simulink library "AFCToolbox2023a"  (R2023a)
settings: Solver=VariableStepAuto  StartTime=0.0  StopTime=10.0  RelTol=1e-3
undefined symbols (not defined in the file or in its folder): AFC5Toolbox_SimuMoudle, AFCToolbox, ax, ay, az, btnSample, C_d, C_dm, C_m, C_t, Control, d, declination_table, dp0, dp1, dp2, dp3, dt, euler_0, g0, I_xyz, inclination_table, J_m, lmd_high, lmd_low, lp_acc_knoise, lp_acc_max, lp_acc_min, lp_acc_seed, lp_GPS_BL_max, lp_GPS_BL_min, lp_GPS_H_max, lp_GPS_H_min, lp_GPS_knoise, lp_GPS_seed, lp_GPS_vel_max, lp_GPS_vel_min, lp_gyro_knoise, lp_gyro_max, lp_gyro_min, lp_gyro_seed, lp_hf_vwind, lp_hs_vwind_interp, lp_kaerorho, lp_kaeroT, lp_kIxyz, lp_kmass, lp_momentx_A0, lp_momentx_Af, lp_momentx_ts, lp_momenty_A0, lp_momenty_Af, lp_momenty_ts, lp_momentz_A0, lp_momentz_Af, lp_momentz_ts, lp_vf_vwind, lp_vs_vwind_interp, lp_vwind_thetax, lp_vwind_thetaz ... (+54)
libraries: $bdroot x104, simulink x75, etargetslib x32, sharedtransform x13, simulink_extras x12, dspstat3 x11, aerolibconvert2 x9, aerolibtransform2 x3, aerolibutil x2, matrix_library x1
(part 1 of 10)
settings Model: Creator=Brolian  LastModifiedBy=zqhkd
settings SolverCC: AlgebraicLoopSolver=TrustRegion
settings DataIOCC: ReturnWorkspaceOutputs=off
settings DebuggingCC: UnconnectedInputMsg=warning  UnconnectedOutputMsg=warning  UnconnectedLineMsg=warning  ArithmeticOperatorsInVariantConditions=warning
settings ModelReferenceCC: EnableRefExpFcnMdlSchedulingChecks=on
settings SFSimCC: SimUseLocalCustomCode=off  CustomCodeUndefinedFunction=UseInterfaceOnly
settings RTWCC: RTWUseLocalCustomCode=off
settings CodeAppCC: StateflowObjectComments=on
settings ConfigComp: CovBoundaryAbsTol=1.0e-5

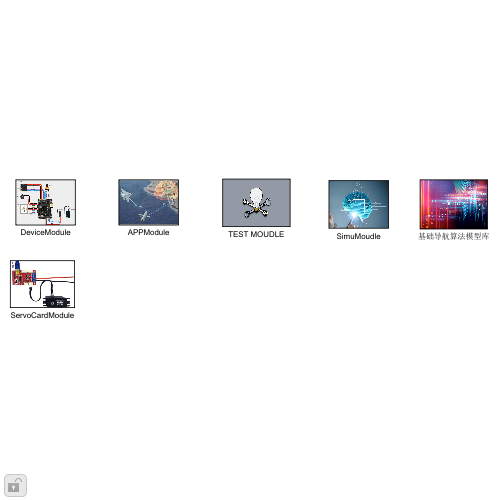
[thumbnail: Simulink's stored preview of the top-level diagram]
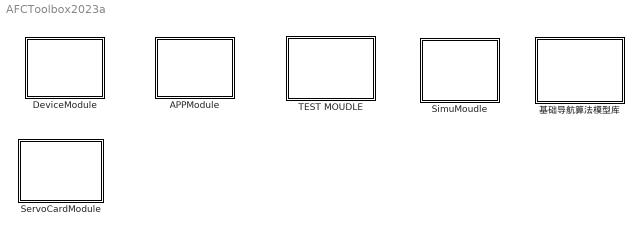
== system AFCToolbox2023a ==
  APPModule : Subsystem
      mask Display: image('AFCApp.png'); % 使用工具条上的 "编辑图像" 进行更改。
  DeviceModule : Subsystem
      mask Display: image('AFCDevice.png'); % 使用工具条上的 "编辑图像" 进行更改。
  ServoCardModule : Subsystem
      mask Display: image('ACEServoCard.png');
  SimuMoudle : Subsystem
      mask Display: image('SimuModule.png'); % 使用工具条上的 "编辑图像" 进行更改。
  TEST MOUDLE : Subsystem
      mask Display: image('TestModule.png'); % 使用工具条上的 "编辑图像" 进行更改。
  基础导航算法模型库 : Subsystem
      mask Display: image('AlgModule.png'); % 使用工具条上的 "编辑图像" 进行更改。

== system AFCToolbox2023a/APPModule ==
  note: ahrs和takeOffLand为V5.03以前
      | 版本库模块，由于Wxyz、Axyz
      | 采用地址传递方式，进行安装正
      | 负号反向处理时已被RTW优化掉
  AFC5StsBit : Subsystem
  RCLimit : S-Function  Priority=4  FunctionName=rcLimitAPI  Parameters=0  SFunctionDeploymentMode=off  EnableBusSupport=off  mask{g_pv=0}
      mask DialogControl Container1 Prompt: AFC-5无人机限幅模块
      mask Display:
      | color('gray');port_label('input',1,'bRCRollLT1000');
      | color('gray');port_label('input',2,'bRCPitchLT1000');
      | color('gray');port_label('input',3,'bRCThrottleEQ0');
      | color('gray');port_label('input',4,'bRCCh3CmdLT1400');
      | color('gray');port_label('input',5,'bRCCh2CmdLT1400');
      | color('gray');port_label('input',6,'bRCCh1CmdLT1600');
      | color('gray');port_label('input',7,'bRCCh0CmdLT1600');
  ahrs : S-Function  Priority=3  Commented=on  FunctionName=ahrsAPI  Parameters=0  SFunctionDeploymentMode=off  EnableBusSupport=off  mask{kp=0.14, ki=0.0087, kp_yaw=0.16, ki_yaw=0.001, dt=0.002, g=9.80665}
      mask prompts: kp "比例控制参数"; ki "积分控制参数"; kp_yaw "比例控制参数"; ki_yaw "积分控制参数"; dt "时间参数"; g "重力加速度"
      mask DialogControl DescGroupVar Prompt: 角速率PI控制参数输入窗口
      mask DialogControl Container2 Prompt: 偏航角速率PI控制参数输入窗口
      mask DialogControl Container3 Prompt: 参数设置窗口
      mask Display:
      | color('gray');port_label('input',1,'Wxyz');
      | color('gray');port_label('input',2,'Axyz');
      | color('gray');port_label('input',3,'HeadAng');
      | color('gray');port_label('input',4,'FastSts');
      | color('gray');port_label('output',1,'dcmAng');
      | color('gray');port_label('output',2,'dcmWxyz');
  ahrsN : S-Function  Priority=3  FunctionName=ahrsNAPI  Parameters=0  SFunctionDeploymentMode=off  EnableBusSupport=off  mask{kp=0.14, ki=0.0087, kp_yaw=0.16, ki_yaw=0.001, dt=0.002, g=9.80665}
      mask prompts: kp "比例控制参数"; ki "积分控制参数"; kp_yaw "比例控制参数"; ki_yaw "积分控制参数"; dt "时间参数"; g "重力加速度"
      mask DialogControl DescGroupVar Prompt: 角速率PI控制参数输入窗口
      mask DialogControl Container2 Prompt: 偏航角速率PI控制参数输入窗口
      mask DialogControl Container3 Prompt: 参数设置窗口
      mask Display:
      | color('gray');port_label('input',1,'Wx /rad/s');
      | color('gray');port_label('input',2,'Wy /rad/s');
      | color('gray');port_label('input',3,'Wz /rad/s');
      | color('gray');port_label('input',4,'Ax /m/s^2');
      | color('gray');port_label('input',5,'Ay /m/s^2');
      | color('gray');port_label('input',6,'Az /m/s^2');
      | color('gray');port_label('input',7,'HeadAng /°');
      | color('gray');port_label('input',8,'FastSts');
      | color('gray');port_label('output',1,'dcmAng /rad');
      | color('gray');port_label('output',2,'dcmWxyz /rad/s');
  altThrottle : S-Function  Priority=4  FunctionName=altThrottleAPI  Parameters=0  SFunctionDeploymentMode=off  EnableBusSupport=off
      mask DialogControl g_pv Prompt: 根据高度通道参数计算油门大小
      mask Display:
      | color('gray');port_label('input',1,'AFC5Sts');
      | color('gray');port_label('input',2,'PosZ');
      | color('gray');port_label('input',3,'VelZ');
      | color('gray');port_label('input',4,'ClimbRate');
      | color('gray');port_label('input',5,'dcmRoll');
      | color('gray');port_label('input',6,'dcmPitch');
      | color('gray');port_label('input',7,'altAccInt');
      | color('gray');port_label('input',8,'posTarZ');
      | color('gray');port_label('input',9,'ThrotHover');
      | color('gray');port_label('output',1,'Throttle');
  altitude : S-Function  Priority=3  FunctionName=altitudeAPI  Parameters=0  SFunctionDeploymentMode=off  EnableBusSupport=off  mask{alt_pos_kp=1.8, pid_alt_rate_kp=8.0, pid_alt_rate_ki=0.1, pid_alt_rate_kd=1.0, pid_alt_rate_imax=800.0, pid_alt_accel_kp=1.36, pid_alt_accel_ki=0.1, pid_alt_accel_kd=0.08, pid_alt_accel_imax=800.0, k1=0.6, k2=0.12, k3=0.008, control_dt=0.002, g=9.80665}
      mask prompts: alt_pos_kp "比例系数"; pid_alt_rate_kp "比例系数"; pid_alt_rate_ki "积分系数"; pid_alt_rate_kd "微分系数"; pid_alt_rate_imax "积分系数最大值"; pid_alt_accel_kp "比例系数"; pid_alt_accel_ki "积分系数"; pid_alt_accel_kd "微分系数"; pid_alt_accel_imax "积分系数最大值"; k1 "位置更新系数"; k2 "速度更新系数"; k3 "加速度更新系数"; control_dt "姿态控制周期"; g "重力加速度"
      mask DialogControl DescGroupVar Prompt: 高度控制参数输入窗口
      mask DialogControl Container2 Prompt: 高度控制回路的位置系数
      mask DialogControl Container3 Prompt: 高度控制回路的速率系数
      mask DialogControl Container4 Prompt: 高度控制回路的加速度系数
      mask DialogControl Container5 Prompt: 高度更新系数输入窗口
      mask DialogControl Container6 Prompt: 参数设置输入窗口
      mask Display:
      | color('gray');port_label('input',1,'AFC5Sts');
      | color('gray');port_label('input',2,'Height /cm');
      | color('gray');port_label('input',3,'dcmRoll /rad');
      | color('gray');port_label('input',4,'dcmPitch /rad');
      | color('gray');port_label('input',5,'Throttle');
      | color('gray');port_label('output',1,'PosZ /cm');
      | color('gray');port_label('output',2,'VelZ /cm/s');
      | color('gray');port_label('output',3,'ThroHover');
  altitudeThrottle : S-Function  Priority=4  FunctionName=altitudeThrottleAPI  Parameters=0  SFunctionDeploymentMode=off  EnableBusSupport=off
      mask DialogControl g_pv Prompt: 根据高度通道参数计算油门大小
      mask Display:
      | color('gray');port_label('input',1,'AFC5Sts');
      | color('gray');port_label('input',2,'PosZ');
      | color('gray');port_label('input',3,'VelZ');
      | color('gray');port_label('input',4,'ClimbRate');
      | color('gray');port_label('input',5,'dcmRoll');
      | color('gray');port_label('input',6,'dcmPitch');
      | color('gray');port_label('input',7,'ThrotHover');
      | color('gray');port_label('output',1,'Throttle');
  attitudePos : S-Function  Priority=3  FunctionName=attitudePosAPI  Parameters=0  SFunctionDeploymentMode=off  EnableBusSupport=off
      mask DialogControl ParameterGroupVar Prompt: 参数
      mask Display:
      | color('gray');port_label('input',1,'rollCmd');
      | color('gray');port_label('input',2,'pitchCmd');
      | color('gray');port_label('input',3,'yawCmd');
      | color('gray');port_label('input',4,'dcmAng');
      | color('gray');port_label('input',5,'Wz');
      | color('gray');port_label('input',6,'AngEfTarZ');
      | color('gray');port_label('output',1,'RateBfTar');
      | color('gray');port_label('output',2,'AngEfTarZ');
  attitudeRate : S-Function  Priority=4  FunctionName=attitudeRateAPI  Parameters=0  SFunctionDeploymentMode=off  EnableBusSupport=off  mask{angle_kp0=8.0, angle_kp1=6.6, angle_kp2=8.0, pid_rate0_kp=0.32, pid_rate0_ki=0.1, pid_rate0_kd=3.5, pid_rate1_kp=0.32, pid_rate1_ki=0.1, pid_rate1_kd=3.5, pid_rate2_kp=0.6, pid_rate2_ki=0.03, pid_rate2_kd=1.5, pid_rate0_imax=500.0, pid_rate1_imax=500.0, pid_rate2_imax=500.0, max0=5000.0, min0=-5000.0, max1=5000.0, min1=-5000.0, max2=4000.0, min2=-4000.0, control_dt=0.002}
      mask prompts: angle_kp0 "横滚角比例系数"; angle_kp1 "俯仰角比例系数"; angle_kp2 "航向角比例系数"; pid_rate0_kp "比例系数"; pid_rate0_ki "积分系数"; pid_rate0_kd "微分系数"; pid_rate1_kp "比例系数"; pid_rate1_ki "积分系数"; pid_rate1_kd "微分系数"; pid_rate2_kp "比例系数"; pid_rate2_ki "积分系数"; pid_rate2_kd "微分系数"; pid_rate0_imax "横滚角速率积分系数最大值"; pid_rate1_imax "俯仰角速率积分系数最大值"; pid_rate2_imax "航向角速率积分系数最大值"; max0 "最大值"; min0 "最小值"; max1 "最大值"; min1 "最小值"; max2 "最大值"; min2 "最小值"; control_dt "姿态控制周期"
      mask DialogControl DescGroupVar Prompt: 姿态角初始化比例系数输入窗口
      mask DialogControl Container2 Prompt: 姿态角速率初始化PI参数输入窗口
      mask DialogControl Container3 Prompt: 横滚角PI参数
      mask DialogControl Container4 Prompt: 俯仰角PI参数
      mask DialogControl Container5 Prompt: 航向角PI参数
      mask DialogControl Container6 Prompt: 姿态角速率积分系数的最大值
      mask DialogControl Container8 Prompt: 姿态角输出限幅设置窗口
      mask DialogControl Container9 Prompt: 横滚角输出限幅
      mask DialogControl Container10 Prompt: 俯仰角输出限幅
      mask DialogControl Container11 Prompt: 航向角输出限幅
      mask DialogControl Container7 Prompt: 参数设置输入窗口
      mask Display:
      | color('gray');port_label('input',1,'AFC5Sts');
      | color('gray');port_label('input',2,'rateBfTar');
      | color('gray');port_label('input',3,'dcmWxyz');
      | color('gray');port_label('output',1,'ServOut');
  ctrlChCmdAPI : S-Function  Priority=3  FunctionName=ctrlChCmdAPI  Parameters=0  SFunctionDeploymentMode=off  EnableBusSupport=off
      mask DialogControl g_pv Prompt: 遥控器SBus原始指令转换为通道指令
      mask Display:
      | color('gray');port_label('input',1,'RCRaw');
      | color('gray');port_label('output',1,'CHCmd');
  flyModeRun : S-Function  Priority=4  FunctionName=flyModeRunAPI  Parameters=0  SFunctionDeploymentMode=off  EnableBusSupport=off
      mask DialogControl g_pv Prompt: 飞行模式调度程序
      mask Display:
      | color('gray');port_label('input',1,'AFCSts');
      | color('gray');port_label('input',2,'PosZ /cm');
      | color('gray');port_label('input',3,'VelZ /cm/s');
      | color('gray');port_label('input',4,'dcmAng /rad');
      | color('gray');port_label('input',5,'dcmWxyz /rad/s');
      | color('gray');port_label('input',6,'ThroHover');
      | color('gray');port_label('input',7,'CHCtrlCmd');
      | color('gray');port_label('output',1,'Throttle');
      | color('gray');port_label('output',2,'RateBfTar');
  getAFCSts : S-Function  Priority=0  FunctionName=getAFCStsAPI  Parameters=g_sampleTime  SFunctionDeploymentMode=off  EnableBusSupport=off  mask{g_sampleTime=0.002}
      mask prompts: g_sampleTime "请输入采样时间："
      mask DialogControl DescGroupVar Prompt: AFC5系统状态
      mask DialogControl g_pv Prompt: 获取AFC5飞控状态，包括:
      mask DialogControl Control2 Prompt: D0：bSystemInitSts,D1：bLandComplete
      mask DialogControl Control3 Prompt: D2：bArmedEnable,D3：bDcmFast
      mask DialogControl Control4 Prompt: D4：bSdCardWriteErr
      mask DialogControl Control5 Prompt: D8--D15：iTaskOverTimeNo
      mask Display: color('gray');port_label('output',1,'AFCSts');
  getRCCmd : S-Function  Commented=on  FunctionName=getRCCmdAPI  Parameters=0  SFunctionDeploymentMode=off  EnableBusSupport=off
      mask DialogControl g_pv Prompt: 通道指令输入模块
      mask Display:
      | color('gray');port_label('output',1,'RollSrvo');
      | color('gray');port_label('output',2,'PitchSrvo');
      | color('gray');port_label('output',3,'YawSrvo');
      | color('gray');port_label('output',4,'Throttle');
      | color('gray');port_label('output',5,'ClimbRate');
  groundProc : S-Function  Priority=4  FunctionName=groundProcAPI  Parameters=0  SFunctionDeploymentMode=off  EnableBusSupport=off
      mask DialogControl ParameterGroupVar Prompt: 参数
      mask Display:
      | color('gray');port_label('input',1,'PosZ');
      | color('gray');port_label('input',2,'dcmAng');
      | color('gray');port_label('input',3,'Wxyz');
      | color('gray');port_label('output',1,'angEfTarZ');
      | color('gray');port_label('output',2,'rateBfTar');
      | color('gray');port_label('output',3,'Throttle');
  initTakeOff : S-Function  Priority=5  FunctionName=initTakeOffAPI  Parameters=0  SFunctionDeploymentMode=off  EnableBusSupport=off
      mask DialogControl g_pv Prompt: 初始化起飞模块
      mask Display:
      | color('gray');port_label('input',1,'PosZ');
      | color('gray');port_label('input',2,'Throttle');
  motorsSlow : S-Function  Commented=on  FunctionName=motorsSlowAPI  Parameters=0  SFunctionDeploymentMode=off  EnableBusSupport=off
      mask DialogControl ParameterGroupVar Prompt: 参数
      mask Display:
      | color('gray');port_label('input',1,'AFC5Sts');
      | color('gray');port_label('input',2,'Throttle');
      | color('gray');port_label('input',3,'inMaxThrottle');
      | color('gray');port_label('output',1,'MaxThrottle');
  outMotorsVal : S-Function  Priority=5  FunctionName=outMotorsValAPI  Parameters=0  SFunctionDeploymentMode=off  EnableBusSupport=off
      mask DialogControl g_pv Prompt: 输出电机电调指令值模块
      mask Display:
      | color('gray');port_label('input',1,'AFC5Sts');
      | color('gray');port_label('input',2,'ServOut');
      | color('gray');port_label('input',3,'Throttle');
      | color('gray');port_label('output',1,'EscVal');
  takeOffLand : S-Function  Priority=5  Commented=on  FunctionName=takeOffLandAPI  Parameters=0  SFunctionDeploymentMode=off  EnableBusSupport=off  mask{RC_Climb_Rate=0}
      mask prompts: RC_Climb_Rate "攀爬速度阈值"
      mask DialogControl g_pv Prompt: 起飞着陆模块
      mask DialogControl Control1 Prompt: (在此添加文本)处理起飞前的IMU校准、遥控解锁，着陆标志判定，电机关机锁定等操作
      mask DialogControl Container2 Prompt: 起飞条件
      mask Display:
      | color('gray');port_label('input',1,'Wxyz');
      | color('gray');port_label('input',2,'Axyz');
      | color('gray');port_label('input',3,'dcmRoll');
      | color('gray');port_label('input',4,'dcmPitch');
      | color('gray');port_label('input',5,'Throttle');
  takeOffLandN : S-Function  Priority=5  FunctionName=takeOffLandNAPI  Parameters=0  SFunctionDeploymentMode=off  EnableBusSupport=off  mask{RC_Climb_Rate=0}
      mask prompts: RC_Climb_Rate "攀爬速度阈值"
      mask DialogControl g_pv Prompt: 起飞着陆模块
      mask DialogControl Control1 Prompt: (在此添加文本)处理起飞前的IMU校准、遥控解锁，着陆标志判定，电机关机锁定等操作
      mask DialogControl Container2 Prompt: 起飞条件
      mask Display:
      | color('gray');port_label('input',1,'Wx');
      | color('gray');port_label('input',2,'Wy');
      | color('gray');port_label('input',3,'Wz');
      | color('gray');port_label('input',4,'Ax');
      | color('gray');port_label('input',5,'Ay');
      | color('gray');port_label('input',6,'Az');
      | color('gray');port_label('input',7,'dcmRoll');
      | color('gray');port_label('input',8,'dcmPitch');
      | color('gray');port_label('input',9,'Throttle');
  u16Toi16 : S-Function  FunctionName=u16Toi16API  Parameters=0  SFunctionDeploymentMode=off  EnableBusSupport=off
      mask DialogControl ParameterGroupVar Prompt: 参数
      mask Display:
      | color('gray');port_label('input',1,'u16');
      | color('gray');port_label('output',1,'i16');
  u32Toi32 : S-Function  FunctionName=u32Toi32API  Parameters=0  SFunctionDeploymentMode=off  EnableBusSupport=off
      mask DialogControl ParameterGroupVar Prompt: 参数
      mask Display:
      | color('gray');port_label('input',1,'u32');
      | color('gray');port_label('output',1,'i32');
  u8Toi8 : S-Function  FunctionName=u8Toi8API  Parameters=0  SFunctionDeploymentMode=off  EnableBusSupport=off
      mask DialogControl ParameterGroupVar Prompt: 参数
      mask Display:
      | color('gray');port_label('input',1,'u8');
      | color('gray');port_label('output',1,'i8');
  updateCd : Subsystem  Commented=on  TreatAsAtomicUnit=on
      settings: MinAlgLoopOccurrences=on  RTWFileNameOpts=Use function name
      mask DialogControl DescGroupVar Prompt: update_cd_values
      mask DialogControl DescTextVar Prompt: 角度角速度单位从弧度转换为度*100

== system AFCToolbox2023a/DeviceModule ==
  AFCTimer : S-Function  Priority=0  FunctionName=sysTimerAPI  Parameters=g_sampleTime,g_comPort,g_instName,g_id  SFunctionDeploymentMode=off  EnableBusSupport=off  mask{g_sampleTime=0.002, g_comPort=6, g_instName=0, g_id=0}
      mask prompts: g_sampleTime "请输入采样时间："
      mask DialogControl DescGroupVar Prompt: AFC-5飞控快速原型时钟模块
      mask DialogControl Control2 Prompt: 本模块能够直接访问AFC-5飞控系统的运行时钟，单位为秒。
      mask Display: color('gray');port_label('output',1,'Tim');
  AdSample : S-Function  Priority=1  FunctionName=adSampleAPI  Parameters=g_sampleTime,g_comPort,g_instName,g_id  SFunctionDeploymentMode=off  EnableBusSupport=off  mask{g_sampleTime=0.01, g_comPort=0, g_instName=0, g_id=0}
      mask prompts: g_sampleTime "请输入采样时间(s)："; g_comPort "COMPORT"
      mask DialogControl DescGroupVar Prompt: 外部电压采集模块
      mask Display:
      | color('gray');port_label('output',1,'Tim /ms');
      | color('gray');port_label('output',2,'I  /A');
      | color('gray');port_label('output',3,'V  /V');
  ComXIn : S-Function  Priority=2  FunctionName=readXXXComAPI  Parameters=g_sampleTime,g_comPort,g_baudRate,g_dataSize,g_dataBits,g_parity,g_stopBits  SFunctionDeploymentMode=off  EnableBusSupport=off  mask{g_sampleTime=0.01, g_comPort=UART4(TTL), g_baudRate=115200, g_dataSize=1, g_dataBits=8, g_parity=0, g_stopBits=1}
      mask prompts: g_sampleTime "采样时间(s)："; g_comPort "请选择串口："; g_baudRate "波特率："; g_dataSize "帧字节数："; g_dataBits "数据位："; g_parity "校验位："; g_stopBits "停止位："
      mask TypeOptions g_comPort: UART4(TTL) | UART5(RS422) | UART6(TTL) | UART7(RS232) | UART8(RS232)
      mask DialogControl DescGroupVar Prompt: 数传串口输入模块
      mask DialogControl g_comPort Tooltip: 该帧类型码范围在80--90，且不同DtCom帧类型码不同
      mask Display:
      | comPort = get_param(gcb, 'g_comPort');
      | color('gray');port_label('output',1,comPort);
  ComXOut : S-Function  Priority=8  FunctionName=writeXXXComAPI  Parameters=g_comPort,g_baudRate,g_outFreq,g_dataBits,g_parity,g_stopBits  SFunctionDeploymentMode=off  EnableBusSupport=off  mask{g_comPort=UART4(TTL), g_baudRate=115200, g_outFreq=1, g_dataBits=8, g_parity=none, g_stopBits=1}
      mask prompts: g_comPort "请选择串口："; g_baudRate "波特率："; g_outFreq "该模块输出帧频次："; g_dataBits "数据位："; g_parity "校验位："; g_stopBits "停止位："
      mask TypeOptions g_comPort: UART4(TTL) | UART5(RS422) | UART6(TTL) | UART7(RS232) | UART8(RS232)
      mask DialogControl DescGroupVar Prompt: 数传串口输出模块
      mask DialogControl g_comPort Tooltip: 串口号
      mask DialogControl g_outFreq Tooltip: 仿真步长整数倍数，即多少个仿真步长输出一次帧数据
      mask Display:
      | comPort = get_param(gcb, 'g_comPort');
      | color('gray');port_label('input',1,comPort);
  DPS310 : S-Function  Priority=1  FunctionName=DPS310API  Parameters=g_sampleTime,g_comPort,g_instName,g_id  SFunctionDeploymentMode=off  EnableBusSupport=off  mask{g_sampleTime=0.01, g_comPort=6, g_instName=0, g_id=0}
      mask prompts: g_sampleTime "采样时间"
      mask DialogControl ParameterGroupVar Prompt: DPS310数字气压计模块
      mask DialogControl Control1 Prompt: 本模块能够读取数字气压计DPS310测得的压力、温度、气压高度
      mask Display:
      | color('gray');port_label('output',1,'Tim /ms');
      | color('gray');port_label('output',2,'Press /Pa');
      | color('gray');port_label('output',3,'Temp /°C');
      | color('gray');port_label('output',4,'BarHeight /m');
  DPS310Rst : Subsystem  Commented=on
  DTComIn : S-Function  Priority=2  FunctionName=readDtComAPI  Parameters=g_sampleTime,g_frameType,g_resFrameNum,g_comPort,g_instName,g_id  SFunctionDeploymentMode=off  EnableBusSupport=off  mask{g_sampleTime=0.01, g_frameType=20, g_resFrameNum=0, g_comPort=6, g_instName=0, g_id=0}
      mask prompts: g_sampleTime "采样时间(s)："; g_frameType "请输入帧类型码："; g_resFrameNum "请输入回令帧次数："
      mask DialogControl DescGroupVar Prompt: 数传串口输入模块
      mask DialogControl g_frameType Tooltip: 该帧类型码范围在80--90，且不同DtCom帧类型码不同
      mask DialogControl g_resFrameNum Tooltip: 当接收到本有效帧后，串口会中止当前发送，改为发送指定回令帧次数后恢复原发送操作，回令帧内容为串口输入时刻的时标和串口输入数据。
      mask DialogControl ChkDtComIn Prompt: 校验输入参数名称
      mask Display:
      | fno = get_param(gcb, 'g_frameType');
      | color('gray');port_label('output',1,'Tim');
      | color('gray');port_label('output',2,['readDT' newline '@' fno]);
  DTComOut : S-Function  Priority=8  FunctionName=writeDtComAPI  Parameters=g_frameType,g_outFreq,g_comPort,g_instName,g_id  SFunctionDeploymentMode=off  EnableBusSupport=off  mask{g_frameType=1, g_outFreq=1, g_comPort=0, g_instName=0, g_id=0}
      mask prompts: g_frameType "自定义帧类型码："; g_outFreq "该模块输出帧频次："
      mask DialogControl DescGroupVar Prompt: 数传串口输出模块
      mask DialogControl g_frameType Tooltip: 该帧类型码取值为1~20，且不同DtCom帧类型码不同
      mask DialogControl g_outFreq Tooltip: 仿真步长整数倍数，即多少个仿真步长输出一次帧数据
      mask DialogControl ChkSignalName Prompt: 校验信号名称
      mask Display:
      | fno = get_param(gcb, 'g_frameType');
      | color('gray');port_label('input',1,['writeDT@' fno]);
  DtOutDevParm : S-Function  FunctionName=DtOutDevParm  Parameters=g_bICM42688EO,g_bICM20602EO,g_bDPSISTEO,g_bGPSEO,g_bRemoterEO  SFunctionDeploymentMode=off  EnableBusSupport=off  mask{g_bICM42688EO=on, g_bICM20602EO=on, g_bDPSISTEO=on, g_bGPSEO=on, g_bRemoterEO=on}
      mask DialogControl ParameterGroupVar Prompt: 参数
  GPS : S-Function  Priority=1  FunctionName=readGpsAPI  Parameters=g_sampleTime,g_gpsDev,g_comPort,g_instName,g_id  SFunctionDeploymentMode=off  EnableBusSupport=off  mask{g_sampleTime=0.1, g_gpsDev=M10 GNSS, g_comPort=6, g_instName=0, g_id=0}
      mask prompts: g_sampleTime "请输入采样时间："; g_gpsDev "请选择GPS设备"
      mask TypeOptions g_gpsDev: M10 GNSS | NANO GNSS
      mask DialogControl DescGroupVar Prompt: GPS接收机信息获取模块
      mask DialogControl Control2 Prompt: 本模块能够直接读取如下GPS信息：Lat -- 纬度，北纬为正（单位：°）；Lon -- 经度，东经为正（单位：°），Alt -- 海拔高度（单位：m）Vx--M10表示正北速度、Nano-D表示ECCF坐标系下Vx（m/s），Vy--M10表示正东速度、Nano-D表示ECCF坐标系下Vy（m/s），Vz--M10表示向上速度、Nano-D表示ECCF坐标系下Vz（m/s），Vgnd -- 地速（单位：m/s），HeadAng -- 真北航向角（单位：°），STS -- GPS状态，stasN--卫星个数, hdop-- 水平精度因子
      mask DialogControl g_gpsDev Tooltip: 请通过下拉菜单选择指定GNSS设备
      mask Display:
      | color('gray');port_label('output',1,'GPSTim /s');
      | color('gray');port_label('output',2,'Lon /°');
      | color('gray');port_label('output',3,'Lat /°');
      | color('gray');port_label('output',4,'Alt /m');
      | color('gray');port_label('output',5,'Vx /m/s');
      | color('gray');port_label('output',6,'Vy /m/s');
      | color('gray');port_label('output',7,'Vz /m/s');
      | color('gray');port_label('output',8,'Vgnd /m/s');
      | color('gray');port_label('output',9,'Head /°');
      | color('gray');port_label('output',10,'Sts');
      | color('gray');port_label('output',11,'stasN');
      | color('gray');port_label('output',12,'hdop');
      | color('gray');port_label('output',13,'AFCTim /ms');
  GPUComIn : S-Function  Commented=on  FunctionName=readGpuComAPI  Parameters=g_frameType,g_sampleTime,g_comPort,g_instName,g_id  SFunctionDeploymentMode=off  EnableBusSupport=off  mask{g_frameType=162, g_sampleTime=0.01, g_comPort=0, g_instName=0, g_id=0}
      mask prompts: g_frameType "请输入帧类型码："; g_sampleTime "采样时间(s)："
      mask DialogControl DescGroupVar Prompt: 模型串口输入模块
      mask Display: color('gray');port_label('output',1,'readGPU');
  GPUComOut : S-Function  Commented=on  FunctionName=writeGpuComAPI  Parameters=g_frameType,g_comPort,g_instName,g_id  SFunctionDeploymentMode=off  EnableBusSupport=off  mask{g_frameType=2, g_comPort=0, g_instName=0, g_id=0}
      mask prompts: g_frameType "请输入帧类型码："
      mask DialogControl DescGroupVar Prompt: GPU串口输出模块
      mask Display: color('gray');port_label('input',1,'writeGPU');
  HiEscCmd : S-Function  Priority=6  FunctionName=hiEscCmdAPI  Parameters=g_chanelNo,g_minPW,g_maxPW,g_comPort,g_instName,g_id  SFunctionDeploymentMode=off  EnableBusSupport=off  mask{g_chanelNo=1, g_minPW=40, g_maxPW=80, g_comPort=6, g_instName=0, g_id=0}
      mask prompts: g_chanelNo "电调指令通道(1--12)："; g_minPW "电调指令最小值："; g_maxPW "电调指令最大值："; g_comPort "串行端口"; g_instName "实例名称"; g_id "ID号"
      mask DialogControl DescGroupVar Prompt: 进行高速电调控制指令参数配置
      mask DialogControl g_minPW Tooltip: 高速电调占空比最小值标称值为40%, 该值可根据实际情况做微小调整
      mask DialogControl g_maxPW Tooltip: 高速电调占空比最大值标称值为80%, 该值可根据实际情况做微小调整
      mask DialogControl Control1 Prompt: 高速电调频率为400Hz，电调指令输入值范围在0~100之间
      mask Display:
      | ch = get_param(gcb, 'g_chanelNo');
      | color('gray');port_label('input',1,['hiEsc#' ch]);
  ICM20602 : S-Function  Priority=0  FunctionName=ICM20602API  Parameters=g_sampleTime,g_GyroRangeSel,g_AcclRangeSel,g_smplrtDiv,g_comPort,g_instName,g_id  SFunctionDeploymentMode=off  EnableBusSupport=off  mask{g_sampleTime=0.002, g_GyroRangeSel=±2000 °/s, g_AcclRangeSel=±8g, g_smplrtDiv=0, g_comPort=6, g_instName=0, g_id=0}
      mask prompts: g_sampleTime "请输入采样时间："; g_GyroRangeSel "陀螺仪测量范围"; g_AcclRangeSel "加计测量范围"; g_smplrtDiv "采样速率分频："
      mask TypeOptions g_GyroRangeSel: ±250 °/s | ±500 °/s | ±1000 °/s | ±2000 °/s
      mask TypeOptions g_AcclRangeSel: ±2g | ±4g | ±8g | ±16g
      mask DialogControl DescGroupVar Prompt: ICM20602惯组接口模块
      mask DialogControl Control2 Prompt: 本模块能够读取ICM20602惯组模块的角速率（rad/s）、过载g（缺省为陀螺仪±250°/s, 加计±2g）
      mask Display:
      | color('gray');port_label('output',1,'Tim /ms');
      | color('gray');port_label('output',2,'Wx /°/s');
      | color('gray');port_label('output',3,'Wy /°/s');
      | color('gray');port_label('output',4,'Wz /°/s');
      | color('gray');port_label('output',5,'Ax / m/s^2');
      | color('gray');port_label('output',6,'Ay / m/s^2');
      | color('gray');port_label('output',7,'Az / m/s^2');
      | color('gray');port_label('output',8,'Temp /°');
  ICM42688 : S-Function  Priority=0  FunctionName=ICM42688API  Parameters=g_sampleTime,g_GyroRangeSel,g_AcclRangeSel,g_antiAliasFilter,g_notchFilter,g_comPort,g_instName,g_id  SFunctionDeploymentMode=off  EnableBusSupport=off  mask{g_sampleTime=0.002, g_GyroRangeSel=±2000 °/s, g_AcclRangeSel=±8g, g_antiAliasFilter=42, g_notchFilter=1449Hz, g_comPort=6, g_instName=0, g_id=0}
      mask prompts: g_sampleTime "请输入采样时间："; g_GyroRangeSel "陀螺仪测量范围"; g_AcclRangeSel "加计测量范围"; g_antiAliasFilter "抗混叠滤波器频率:"; g_notchFilter "限波器带宽:"; g_comPort "串口号"; g_instName "实例名"; g_id "ID号"
      mask TypeOptions g_GyroRangeSel: ±2000 °/s | ±1000°/s | ±500 °/s | ±250 °/s | ±125 °/s | ±62.5°/s | ±31.25°/s | ±15.625°/s
      mask TypeOptions g_AcclRangeSel: ±16g | ±8g | ±4g | ±2g
      mask TypeOptions g_antiAliasFilter: 禁止 | 42 Hz | 84 Hz | 126 Hz | 170 Hz | 213 Hz | 258 Hz | 303 Hz | 348 Hz | 394 Hz | 441 Hz | 488 Hz | 536 Hz | 585 Hz | 634 Hz | 684 Hz | 734 Hz | 785 Hz | 837 Hz | 890 Hz | 943 Hz | 997 Hz | 1051Hz | 1107Hz | 1163Hz | 1220Hz | 1277Hz | 1336Hz | 1395Hz | 1454Hz | 1515Hz | 1577Hz | 1639Hz | 1702Hz | 1766Hz | 1830Hz | 1896Hz | 1962Hz | 2029Hz | 2097Hz | 2166Hz | 2235Hz | 2306Hz | 2377Hz | 2449Hz | 2522Hz | 2596Hz | 2671Hz | 2746Hz | 2823Hz | 2900Hz | 2978Hz | 3057Hz | 3137Hz | 3217Hz | 3299Hz | 3381Hz | 3464Hz | 3548Hz | 3633Hz | 3718Hz | 3805Hz | 3892Hz | 3979Hz
      mask TypeOptions g_notchFilter: 禁止 | 1449Hz | 680  Hz | 329  Hz | 162  Hz | 80  Hz | 40  Hz | 20  Hz | 10  Hz
      mask DialogControl DescGroupVar Prompt: ICM42688惯组接口模块
      mask DialogControl Control2 Prompt: 本模块能够读取ICM42688惯组模块的角速率（rad/s）、过载g（缺省为陀螺仪±2000°/s, 加计±16g）
      mask DialogControl g_antiAliasFilter Tooltip: 可配置抗混叠滤波器频率为42~3979Hz
      mask DialogControl g_notchFilter Tooltip: 可配置限波器频率为10~1449Hz
      mask Display:
      | color('gray');port_label('output',1,'Tim /ms');
      | color('gray');port_label('output',2,'Wx /rad/s');
      | color('gray');port_label('output',3,'Wy /rad/s');
      | color('gray');port_label('output',4,'Wz /rad/s');
      | color('gray');port_label('output',5,'Ax /m/s^2');
      | color('gray');port_label('output',6,'Ay / m/s^2');
      | color('gray');port_label('output',7,'Az / m/s^2');
      | color('gray');port_label('output',8,'Temp /°');
  IST8310 : S-Function  Priority=1  FunctionName=IST8310API  Parameters=g_sampleTime,g_comPort,g_instName,g_id  SFunctionDeploymentMode=off  EnableBusSupport=off  mask{g_sampleTime=0.01, g_comPort=0, g_instName=0, g_id=0}
      mask prompts: g_sampleTime "请输入采样时间："
      mask DialogControl ParameterGroupVar Prompt: IST8310地磁传感器接口模块
      mask DialogControl Control1 Prompt: 本模块能够读取地磁传感器IST8310测得的三轴地磁强度（单位：uT）
      mask Display:
      | color('gray');port_label('output',1,'Tim /ms');
      | color('gray');port_label('output',2,'MagX /uT');
      | color('gray');port_label('output',3,'MagY /uT');
      | color('gray');port_label('output',4,'MagZ /uT');
      | color('gray');port_label('output',5,'HeadAng /°');
  LedBit : S-Function  Priority=6  FunctionName=ledBitAPI  Parameters=g_chanelNo,g_comPort,g_instName,g_id  SFunctionDeploymentMode=off  EnableBusSupport=off  mask{g_chanelNo=绿色指示灯, g_comPort=0, g_instName=0, g_id=0}
      mask prompts: g_chanelNo "指示灯："
      mask TypeOptions g_chanelNo: 黄色指示灯 | 绿色指示灯 | 蓝色指示灯 | 红色指示灯
      mask DialogControl DescGroupVar Prompt: 选择LED指示灯
      mask DialogControl g_chanelNo Tooltip: 请通过下拉菜单选择指定指示灯
      mask Display:
      | ch = get_param(gcb, 'g_chanelNo');
      | color('gray');port_label('input',1,ch);
      | %color('blue');
      | %disp(['MonitorIP' newline ch]);
      | %disp([newline newline ch]);
  LedGroup : S-Function  Priority=7  FunctionName=ledGroupAPI  Parameters=g_frameType,g_comPort,g_instName,g_id  SFunctionDeploymentMode=off  EnableBusSupport=off  mask{g_frameType=0, g_comPort=6, g_instName=0, g_id=0}
      mask prompts: g_frameType "请输入帧类型码："
      mask DialogControl DescGroupVar Prompt: LED颜色与系统状态指示模块
      mask Display:
      | color('gray');port_label('input',1,'Fly(Y)');
      | color('gray');port_label('input',2,'Test(G)');
      | color('gray');port_label('input',3,'DL(B)');
      | color('gray');port_label('input',4,'Err(R)');
  LowEscCmd : S-Function  Priority=6  FunctionName=lowEscCmdAPI  Parameters=g_chanelNo,g_minPW,g_maxPW,g_comPort,g_instName,g_id  SFunctionDeploymentMode=off  EnableBusSupport=off  mask{g_chanelNo=1, g_minPW=5.6, g_maxPW=11.45, g_comPort=6, g_instName=0, g_id=0}
      mask prompts: g_chanelNo "电调指令通道(1--12)："; g_minPW "电调指令最小值："; g_maxPW "电调指令最大值："; g_comPort "串行端口"; g_instName "实例名称"; g_id "ID号"
      mask DialogControl DescGroupVar Prompt: 进行低速电调控制指令参数配置
      mask DialogControl g_minPW Tooltip: 低速电调占空比最小值标称值为2.5%, 该值可根据实际情况做微小调整
      mask DialogControl g_maxPW Tooltip: 低速电调占空比最大值标称值为12.5%, 该值可根据实际情况做微小调整
      mask DialogControl Control1 Prompt: 低速电调频率为50Hz，电调指令输入值范围在0~100之间
      mask Display:
      | ch = get_param(gcb, 'g_chanelNo');
      | color('gray');port_label('input',1,['loEsc#' ch]);
  MS5525 : S-Function  Priority=1  FunctionName=MS5525API  Parameters=g_sampleTime,g_comPort,g_instName,g_id  SFunctionDeploymentMode=off  EnableBusSupport=off  mask{g_sampleTime=0.01, g_comPort=6, g_instName=0, g_id=0}
      mask prompts: g_sampleTime "采样时间"
      mask DialogControl ParameterGroupVar Prompt: MS5525空速计模块
      mask DialogControl Control1 Prompt: 本模块能够读取空速计MS5525测得的动压、温度和指示空速
      mask Display:
      | color('gray');port_label('output',1,'Tim /ms');
      | color('gray');port_label('output',2,'DifP /Pa');
      | color('gray');port_label('output',3,'Temp /°C');
      | color('gray');port_label('output',4,'IAS /m/s');
  MS5525Bias : S-Function  Priority=6  FunctionName=calMS5525BiasAPI  Parameters=g_sampleTime,g_comPort,g_instName,g_id  SFunctionDeploymentMode=off  EnableBusSupport=off  mask{g_sampleTime=2, g_comPort=0, g_instName=0, g_id=0}
      mask prompts: g_sampleTime "空速计校准采样时间（单位：秒）"
      mask DialogControl DescGroupVar Prompt: 空速计校准采样时间
      mask DialogControl g_sampleTime Tooltip: 请通过下拉菜单选择指定指示灯
      mask DialogControl Control1 Prompt: 【输入端口Calib接收到一个上升沿信号时执行校准操作】
      mask Display: color('gray');port_label('input',1,'Calib');
  PWMSample : S-Function  Priority=1  FunctionName=pwmSampleAPI  Parameters=g_sampleTime,g_comPort,g_instName,g_id  SFunctionDeploymentMode=off  EnableBusSupport=off  mask{g_sampleTime=0.01, g_comPort=6, g_instName=0, g_id=0}
      mask prompts: g_sampleTime "请输入采样时间(s)："
      mask DialogControl DescGroupVar Prompt: 舵系统角度采集模块
      mask DialogControl Control1 Prompt: 规定采样输出参数为-100~+100之间的值，其对应PWM 400Hz信号的高电平脉宽1ms~2ms, 占空比40%--80%
      mask Display:
      | color('gray');port_label('output',1,'Ch1');
      | color('gray');port_label('output',2,'Ch2');
  PressScanner : S-Function  Priority=1  FunctionName=pressScanAPI  Parameters=g_sampleTime,g_comPort,g_instName,g_id  SFunctionDeploymentMode=off  EnableBusSupport=off  mask{g_sampleTime=0.1, g_comPort=6, g_instName=0, g_id=0}
      mask prompts: g_sampleTime "请输入采样时间："
      mask DialogControl DescGroupVar Prompt: 压力扫描阀模块
      mask DialogControl Control2 Prompt: 本模块能够实时采集32通道压强信号。
      mask Display:
      | color('gray');port_label('output',1,'CH0 /kPa');
      | color('gray');port_label('output',2,'CH1 /kPa');
      | color('gray');port_label('output',3,'CH2 /kPa');
      | color('gray');port_label('output',4,'CH3 /kPa');
      | color('gray');port_label('output',5,'CH4 /kPa');
      | color('gray');port_label('output',6,'CH5 /kPa');
      | color('gray');port_label('output',7,'CH6 /kPa');
      | color('gray');port_label('output',8,'CH7 /kPa');
      | color('gray');port_label('output',9,'CH8 /kPa');
      | color('gray');port_label('output',10,'CH9 /kPa');
      | color('gray');port_label('output',11,'CH10 /kPa');
      | color('gray');port_label('output',12,'CH11 /kPa');
      | color('gray');port_label('output',13,'CH12 /kPa');
      | color('gray');port_label('output',14,'CH13 /kPa');
      | color('gray');port_label('output',15,'CH14 /kPa');
      | color('gray');port_label('output',16,'CH15 /kPa');
      | color('gray');port_label('output',17,'CH16 /kPa');
      | color('gray');port_label('output',18,'CH17 /kPa');
      | color('gray');port_label('output',19,'CH18 /kPa');
      | color('gray');port_label('output',20,'CH19 /kPa');
      | color('gray');port_label('output',21,'CH20 /kPa');
      | color('gray');port_label('output',22,'CH21 /kPa');
      | color('gray');port_label('output',23,'CH22 /kPa');
      | color('gray');port_label('output',24,'CH23 /kPa');
      | color('gray');port_label('output',25,'CH24 /kPa');
      | color('gray');port_label('output',26,'CH25 /kPa');
      | color('gray');port_label('output',27,'CH26 /kPa');
      | color('gray');port_label('output',28,'CH27 /kPa');
      | color('gray');port_label('output',29,'CH28 /kPa');
      | color('gray');port_label('output',30,'CH29 /kPa');
      | color('gray');port_label('output',31,'CH30 /kPa');
      | color('gray');port_label('output',32,'CH31 /kPa');
      | color('gray');port_label('output',33,'AFCTim /ms');
  SBusCmd : S-Function  Priority=0  FunctionName=readSBusCmdAPI  Parameters=g_sampleTime,g_chanelNo,g_comPort,g_instName,g_id  SFunctionDeploymentMode=off  EnableBusSupport=off  mask{g_sampleTime=0.002, g_chanelNo=1, g_comPort=6, g_instName=0, g_id=0}
      mask prompts: g_sampleTime "请输入采样时间(s)："; g_chanelNo "通道号："
      mask DialogControl DescGroupVar Prompt: 遥控指令采集模块
      mask DialogControl g_chanelNo Tooltip: 通道16为遥控指令刷新标志，其值为0表示未更新，1表示更新。
      mask DialogControl Control1 Prompt: 遥控器采集原始值，各通道原始值范围为352(0x160)--1695(0x69F)，中位1024(0x400)。
      mask Display: color('gray');port_label('output',1,'Cmd');
  SeqInst : S-Function  Priority=6  FunctionName=seqCtrlAPI  Parameters=g_chanelNo,g_comPort,g_instName,g_id  SFunctionDeploymentMode=off  EnableBusSupport=off  mask{g_chanelNo=时序指令1, g_comPort=0, g_instName=0, g_id=0}
      mask prompts: g_chanelNo "时序指令通道号："
      mask TypeOptions g_chanelNo: 时序指令1 | 时序指令2 | 时序指令3 | 时序指令4 | 时序指令5 | 时序指令6 | 时序指令7 | 时序指令8
      mask DialogControl DescGroupVar Prompt: 选择时序控制指令
      mask DialogControl g_chanelNo Tooltip: 请通过下拉菜单选择指定指示灯
      mask Display:
      | %color('gray');port_label('input',1,'S');
      | chNo = get_param(gcbh, 'g_chanelNo');
      | disp(chNo);
  SimuComIn : S-Function  Priority=2  FunctionName=readSimuComAPI  Parameters=g_sampleTime,g_frameType,g_resFrameNum,g_comPort,g_instName,g_id  SFunctionDeploymentMode=off  EnableBusSupport=off  mask{g_sampleTime=0.01, g_frameType=80, g_resFrameNum=0, g_comPort=6, g_instName=0, g_id=0}
      mask prompts: g_sampleTime "采样时间(s)："; g_frameType "请输入帧类型码："; g_resFrameNum "请输入回令帧帧数："
      mask DialogControl DescGroupVar Prompt: 仿真串口输入模块
      mask DialogControl g_frameType Tooltip: 自定义帧类型码范围在1--20，且不同SimuCom帧类型码不同
      mask DialogControl g_resFrameNum Tooltip: 当接收到本有效帧后，串口会中止当前发送，改为发送指定回令帧次数后恢复原发送操作，回令帧内容为串口输入时刻的时标和串口输入数据。
      mask Display:
      | color('gray');port_label('output',1,'Tim');
      | color('gray');port_label('output',2,'readSimu');
  SimuComOut : S-Function  Priority=8  FunctionName=writeSimuComAPI  Parameters=g_frameType,g_outFreq,g_comPort,g_instName,g_id  SFunctionDeploymentMode=off  EnableBusSupport=off  mask{g_frameType=1, g_outFreq=1, g_comPort=0, g_instName=0, g_id=0}
      mask prompts: g_frameType "请输入帧类型码："; g_outFreq "该模块输出帧频次："
      mask DialogControl DescGroupVar Prompt: 仿真串口输出模块
      mask DialogControl g_frameType Tooltip: 该帧类型码取值为1~20，且不同SimuCom帧类型码不同
      mask DialogControl g_outFreq Tooltip: 仿真步长整数倍数，即多少个仿真步长输出一次帧数据
      mask Display: color('gray');port_label('input',1,'writeSimu');
  SrvoCmd : S-Function  Commented=on  FunctionName=srvoCmdAPI  Parameters=g_chanelNo,g_minPW,g_maxPW,g_comPort,g_instName,g_id  SFunctionDeploymentMode=off  EnableBusSupport=off  mask{g_chanelNo=1, g_minPW=40, g_maxPW=76.72, g_comPort=0, g_instName=0, g_id=0}
      mask prompts: g_chanelNo "舵机指令通道(1--12)："; g_minPW "最小开度占空比%："; g_maxPW "最大开度占空比%："
      mask DialogControl DescGroupVar Prompt: 进行舵机控制指令参数配置
      mask DialogControl g_minPW Tooltip: 值在2--90之间，需要用示波器监测
      mask DialogControl g_maxPW Tooltip: 值在2--90之间，需要用示波器监测
      mask DialogControl Control1 Prompt: 舵机指令输入值范围为-90~+90
      mask Display: color('gray');port_label('input',1,'Inst');
  StartSts : S-Function  Priority=2  AncestorBlock=AFCToolbox/btnSample  FunctionName=startStsSampleAPI  Parameters=g_sampleTime,g_comPort,g_instName,g_id  SFunctionDeploymentMode=off  EnableBusSupport=off  mask{g_sampleTime=0.01, g_comPort=0, g_instName=0, g_id=0}
      mask prompts: g_sampleTime "请输入采样时间(s)："
      mask DialogControl DescGroupVar Prompt: 启动开关或同步开关状态采集模块
      mask Display: color('gray');port_label('output',1,'Start');
  TF03 : S-Function  Priority=1  FunctionName=TOF03API  Parameters=g_sampleTime,g_slideNum,g_comPort,g_instName,g_id  SFunctionDeploymentMode=off  EnableBusSupport=off  mask{g_sampleTime=0.01, g_slideNum=1, g_comPort=0, g_instName=0, g_id=0}
      mask prompts: g_sampleTime "请输入采样时间(s)："; g_slideNum "滑动滤波数据点数："; g_comPort "COMPORT"
      mask DialogControl DescGroupVar Prompt: 激光测距TF03模块
      mask DialogControl Control1 Prompt: 该模块输出激光测距值，最大测量范围0.1m--100m/180m, 测量精度10cm，和信号强度，正常测距的信号强度值范围为40--1200，低于40测距超量程
      mask Display:
      | color('gray');port_label('output',1,'Tim /ms');
      | color('gray');port_label('output',2,'Dist /m');
      | color('gray');port_label('output',3,'Strg');
  TaskScheduler : S-Function  Priority=2  FunctionName=taskSchedulerAPI  Parameters=task01Period,task02Period,task03Period  SFunctionDeploymentMode=off  EnableBusSupport=off  mask{task01Period=10, task02Period=0, task03Period=0}
      mask prompts: task01Period "Task01高优先级任务周期(ms)："; task02Period "Task02高优先级任务周期(ms)："; task03Period "Task03高优先级任务周期(ms)："
      mask DialogControl DescGroupVar Prompt: 任务调度模块
      mask DialogControl task01Period Tooltip: 设置为0时将关闭该任务线程
      mask DialogControl task02Period Tooltip: 设置为0时将关闭该任务线程
      mask DialogControl task03Period Tooltip: 设置为0时将关闭该任务线程
      mask Display: color('gray');port_label('output',1,'Task');
  TempratureScanner : S-Function  Priority=1  FunctionName=tempratureScanAPI  Parameters=g_sampleTime,g_comPort,g_instName,g_id  SFunctionDeploymentMode=off  EnableBusSupport=off  mask{g_sampleTime=0.1, g_comPort=6, g_instName=0, g_id=0}
      mask prompts: g_sampleTime "请输入采样时间："
      mask DialogControl DescGroupVar Prompt: 温度扫描阀模块
      mask DialogControl Control2 Prompt: 本模块能够实时采集12通道温度信号。
      mask Display:
      | color('gray');port_label('output',1,'CH0 /°C');
      | color('gray');port_label('output',2,'CH1 /°C');
      | color('gray');port_label('output',3,'CH2 /°C');
      | color('gray');port_label('output',4,'CH3 /°C');
      | color('gray');port_label('output',5,'CH4 /°C');
      | color('gray');port_label('output',6,'CH5 /°C');
      | color('gray');port_label('output',7,'CH6 /°C');
      | color('gray');port_label('output',8,'CH7 /°C');
      | color('gray');port_label('output',9,'CH8 /°C');
      | color('gray');port_label('output',10,'CH9 /°C');
      | color('gray');port_label('output',11,'CH10 /°C');
      | color('gray');port_label('output',12,'CH11 /°C');
      | color('gray');port_label('output',13,'AFCTim /ms');
  USBDisk : S-Function  Priority=8  FunctionName=writeUSBDiskAPI  Parameters=g_taskName,g_varName,g_outFreq,g_comPort,g_instName,g_id  SFunctionDeploymentMode=off  EnableBusSupport=off  mask{g_taskName=F, g_varName=x1,x2,x3,x4, g_outFreq=1, g_comPort=0, g_instName=0, g_id=0}
      mask prompts: g_taskName "请输入任务名称："; g_varName "请输入用逗号分开的所有变量名称："; g_outFreq "请输入写入频次："
      mask DialogControl DescGroupVar Prompt: USB DISK存盘模块
      mask DialogControl g_taskName Tooltip: 任务名长度不超过8个字符
      mask DialogControl g_varName Tooltip: 该名称为数据首行的抬头
      mask DialogControl g_outFreq Tooltip: 写入频次应该为仿真步长整数倍，如果为0表示不写入
      mask Display: color('gray');port_label('input',1,'writeDisk');
  UavId : S-Function  Priority=0  FunctionName=uavIdAPI  Parameters=g_sampleTime,g_comPort,g_instName,g_id  SFunctionDeploymentMode=off  EnableBusSupport=off  mask{g_sampleTime=0.002, g_comPort=6, g_instName=0, g_id=0}
      mask prompts: g_sampleTime "请输入采样时间："
      mask DialogControl DescGroupVar Prompt: AFC-5飞控组件ID获取模块
      mask DialogControl Control2 Prompt: 本模块能够直接读取AFC-5飞控组件ID号
      mask Display: color('gray');port_label('output',1,'uavID');
  UserEscCmd : S-Function  Priority=6  FunctionName=userEscCmdAPI  Parameters=g_chanelNo,g_minPW,g_maxPW,g_userFreq,g_comPort,g_instName,g_id  SFunctionDeploymentMode=off  EnableBusSupport=off  mask{g_chanelNo=1, g_minPW=40, g_maxPW=80, g_userFreq=20000, g_comPort=6, g_instName=0, g_id=0}
      mask prompts: g_chanelNo "电调指令通道(1--12)："; g_minPW "电调指令最小值："; g_maxPW "电调指令最大值："; g_userFreq "用户自定义电调频率(40--40000Hz)"; g_comPort "串行端口"; g_instName "实例名称"; g_id "ID号"
      mask DialogControl DescGroupVar Prompt: 进行高速电调控制指令参数配置
      mask DialogControl g_minPW Tooltip: 高速电调占空比最小值标称值为40%, 该值可根据实际情况做微小调整
      mask DialogControl g_maxPW Tooltip: 高速电调占空比最大值标称值为80%, 该值可根据实际情况做微小调整
      mask DialogControl Control1 Prompt: 电调指令输入值范围在0~100之间，而电调频率为用户定义频率，设置时需要注意以下事项：
      mask DialogControl Control2 Prompt: 【注意事项】第1、2电调通道的PWM频率必须相同；
      mask DialogControl Control3 Prompt: 第3 ~ 6共4个电调通道的PWM频率必须相同；
      mask DialogControl Control4 Prompt: 第7 ~ 10共4个电调通道的PWM频率必须相同；
      mask DialogControl Control5 Prompt: 第11、12两个通道的PWM频率可独立设置。
      mask Display:
      | ch = get_param(gcb, 'g_chanelNo');
      | color('gray');port_label('input',1,['userEsc#' ch]);
  WLanIn : S-Function  Priority=2  FunctionName=readWLanAPI  Parameters=g_sampleTime,g_ipAddress,g_localIpAddress,g_iPort,g_dataSize  SFunctionDeploymentMode=off  EnableBusSupport=off  mask{g_sampleTime=0.01, g_ipAddress=192.168.1.18, g_localIpAddress=192.168.1.11, g_iPort=8080, g_dataSize=1}
      mask prompts: g_sampleTime "采样时间(s)："; g_ipAddress "目标(监测网口)IP地址："; g_localIpAddress "本机(控制器)IP地址："; g_iPort "端口号："; g_dataSize "接收字节数："
      mask DialogControl DescGroupVar Prompt: 数传串口输入模块
      mask DialogControl g_ipAddress Tooltip: 该帧类型码范围在80--90，且不同DtCom帧类型码不同
      mask Display:
      | %color('gray');port_label('output',1,'readLan');
      | ip   = get_param(gcb, 'g_ipAddress');
      | localIp   = get_param(gcb, 'g_localIpAddress');
      | port = get_param(gcb, 'g_iPort');
      | color('gray');
      | disp(['From:' ip newline 'Local:' localIp newline 'PortNo: ' port]);
  WLanOut : S-Function  Priority=8  FunctionName=writeWLanAPI  Parameters=g_ipAddress,g_localIpAddress,g_iPort,g_outFreq  SFunctionDeploymentMode=off  EnableBusSupport=off  mask{g_ipAddress=192.168.1.18, g_localIpAddress=192.168.1.11, g_iPort=8080, g_outFreq=1}
      mask prompts: g_ipAddress "目标(监测网口)IP地址："; g_localIpAddress "本机(控制器网口)IP地址："; g_iPort "发送端口号："; g_outFreq "该模块输出帧频次："
      mask DialogControl DescGroupVar Prompt: 数传串口输出模块
      mask DialogControl g_ipAddress Tooltip: 串口号
      mask DialogControl g_outFreq Tooltip: 仿真步长整数倍数，即多少个仿真步长输出一次帧数据
      mask Display:
      | %color('gray');port_label('input',1,'writeLan');
      | ip   = get_param(gcb, 'g_ipAddress');
      | localIp   = get_param(gcb, 'g_localIpAddress');
      | port = get_param(gcb, 'g_iPort');
      | color('gray');
      | disp(['To:  ' ip newline 'Loc:' localIp newline 'PortNo: ' port]);
  dshotEscCmd : S-Function  Priority=6  FunctionName=dshotEscCmdAPI  Parameters=g_escType,g_chanelNo,g_comPort,g_instName,g_id  SFunctionDeploymentMode=off  EnableBusSupport=off  mask{g_escType=DShot600, g_chanelNo=1, g_comPort=6, g_instName=0, g_id=0}
      mask prompts: g_escType "DShot电调类型"; g_chanelNo "电调指令通道(1--12)："; g_comPort "串行端口"; g_instName "实例名称"; g_id "ID号"
      mask TypeOptions g_escType: DShot100 | DShot150 | DShot300 | DShot600 | DShot1200
      mask DialogControl DescGroupVar Prompt: 进行DShot电调控制指令参数配置
      mask DialogControl Control1 Prompt: DShot电调指令输入值范围在0~100之间
      mask Display:
      | ch = get_param(gcb, 'g_chanelNo');
      | color('gray');port_label('input',1,['dShot#' ch]);

== system AFCToolbox2023a/ServoCardModule ==
  LED Control : Subsystem
  XSimPack : Subsystem  mask{frameSender=0, frameType=5}
      mask DialogControl ParameterGroupVar Prompt: 发送方(dec)
      mask DialogControl Container3 Prompt: 帧类型码(dec)
  XSimUnPack : Subsystem
  XSrvoCmd : Subsystem
  XSrvoSamp : Subsystem
